simulink model "modelemoteur"  (R2024b)
settings: Solver=VariableStepAuto  StartTime=0.0  StopTime=3000  RelTol=1e-3
settings Model: Creator=geii  LastModifiedBy=geii

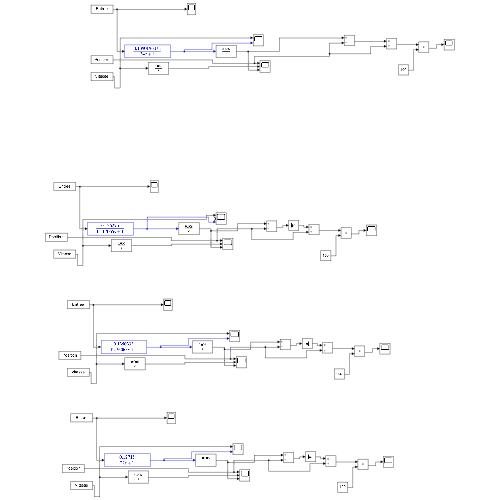
[thumbnail: Simulink's stored preview of the top-level diagram]
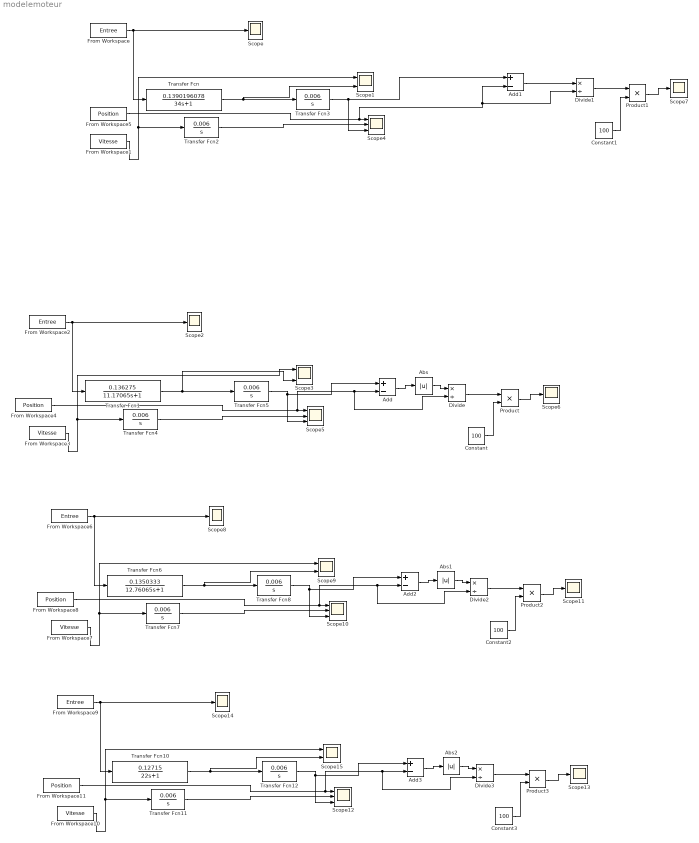
== system modelemoteur ==
  Abs : Abs  SaturateOnIntegerOverflow=off
  Abs1 : Abs  SaturateOnIntegerOverflow=off
  Abs2 : Abs  SaturateOnIntegerOverflow=off
  Add{,1..3} (4 alike) : Sum  Inputs=+-
  Constant{,1..3} (4 alike) : Constant  Value=100
  Divide{,1..3} (4 alike) : Product  Inputs=*/
  From Workspace{,2,6,9} (4 alike) : FromWorkspace  VariableName=Entree  SampleTime=1
  From Workspace{1,3,7,10} (4 alike) : FromWorkspace  VariableName=Vitesse
  From Workspace{4..5,8,11} (4 alike) : FromWorkspace  VariableName=Position
  Product{,1..3} (4 alike) : Product
  Scope{,2,6..8,11,13..14} (8 alike) : Scope
  Scope1 : Scope  NumInputPorts=2
  Scope{3..5,10,12} (5 alike) : Scope  NumInputPorts=3
  Scope15 : Scope  NumInputPorts=2
  Scope9 : Scope  NumInputPorts=2
  Transfer Fcn : TransferFcn  Numerator=[0.1390196078]  Denominator=[34 1]
  Transfer Fcn1 : TransferFcn  Numerator=[0.136275]  Denominator=[11.17065 1]
  Transfer Fcn10 : TransferFcn  Numerator=[0.12715]  Denominator=[22 1]
  Transfer Fcn{2..5,7..8,11..12} (8 alike) : TransferFcn  Numerator=[0.006]  Denominator=[1 0]
  Transfer Fcn6 : TransferFcn  Numerator=[0.1350333]  Denominator=[12.76065 1]
  wires:
  From Workspace/1 -> Transfer Fcn/1, Scope/1
  From Workspace1/1 -> Transfer Fcn2/1, Scope1/1
  Transfer Fcn/1 -> Scope1/2, Transfer Fcn3/1
  Transfer Fcn2/1 -> Scope4/2
  From Workspace4/1 -> Divide/2, Add/2, Scope5/1
  Transfer Fcn5/1 -> Scope5/3, Add/1
  From Workspace3/1 -> Transfer Fcn4/1, Scope3/1
  From Workspace2/1 -> Transfer Fcn1/1, Scope2/1
  Transfer Fcn4/1 -> Scope5/2
  Transfer Fcn1/1 -> Scope3/3, Transfer Fcn5/1
  Divide/1 -> Product/1
  Product/1 -> Scope6/1
  Constant/1 -> Product/2
  Constant1/1 -> Product1/2
  From Workspace5/1 -> Add1/2, Divide1/2, Scope4/1
  Transfer Fcn3/1 -> Add1/1, Scope4/3
  Divide1/1 -> Product1/1
  Add1/1 -> Divide1/1
  Product1/1 -> Scope7/1
  Add/1 -> Abs/1
  Abs/1 -> Divide/1
  Product2/1 -> Scope11/1
  Add2/1 -> Abs1/1
  From Workspace6/1 -> Transfer Fcn6/1, Scope8/1
  Transfer Fcn7/1 -> Scope10/2
  Transfer Fcn6/1 -> Scope9/2, Transfer Fcn8/1
  Constant2/1 -> Product2/2
  Abs1/1 -> Divide2/1
  Divide2/1 -> Product2/1
  From Workspace7/1 -> Transfer Fcn7/1, Scope9/1
  Transfer Fcn8/1 -> Scope10/3, Add2/1
  From Workspace8/1 -> Divide2/2, Add2/2, Scope10/1
  From Workspace11/1 -> Divide3/2, Add3/2, Scope12/1
  Transfer Fcn12/1 -> Scope12/3, Add3/1
  Transfer Fcn11/1 -> Scope12/2
  Abs2/1 -> Divide3/1
  Transfer Fcn10/1 -> Scope15/2, Transfer Fcn12/1
  From Workspace9/1 -> Transfer Fcn10/1, Scope14/1
  Constant3/1 -> Product3/2
  Divide3/1 -> Product3/1
  Product3/1 -> Scope13/1
  Add3/1 -> Abs2/1
  From Workspace10/1 -> Transfer Fcn11/1, Scope15/1
